simulink model "q_aero_2dof_pid_control_new"  (R2025a)
settings: Solver=ode1  StartTime=0.0  StopTime=Tend  FixedStep=0.002  RelTol=1e-3  EnableMultiTasking=on
PreLoadFcn:
  | quanser_aero_pd_design;
values from neighbouring files (symbols this model uses):
  kp_p = P.Jp*wp^2 - P.Ksp    [decoupled_pd_AERO.m]    (also in decoupled_pd_volt_torque.m = P.Jp*wn^2 - P.Ksp; figures_pd_presentation_AERO.m = P.Jp*wn^2 - P.Ksp; plot_decoupled_pd_tests_AERO.m = P.Jp*wn^2 - P.Ksp; setup_decoupled_pd_simulink.m = P.Jp*wn^2 - P.Ksp)
  kp_y = P.Jy*wy^2    [decoupled_pd_AERO.m]    (also in decoupled_pd_volt_torque.m = P.Jy*wn^2; figures_pd_presentation_AERO.m = P.Jy*wn^2; plot_decoupled_pd_tests_AERO.m = P.Jy*wn^2; setup_decoupled_pd_simulink.m = P.Jy*wn^2)
  Ksp = P.Ksp    [decoupled_pd_volt_torque.m]    (also in setup_decoupled_pd_simulink.m)
  W = inv(Wdec)    [decoupled_pd_AERO.m]    (also in decoupled_pd_volt_torque.m = inv([P.Kpp P.Kpy; P.Kyp P.Kyy]); setup_decoupled_pd_simulink.m = inv(Bt))
libraries: simulink_extras x4, quarc_library x3, quanser_aero x1
settings Model: SimulationMode=external  ExtModeTrigDuration=15000  Creator=MLevis  LastModifiedBy=e82540u
settings SolverCC: AlgebraicLoopSolver=TrustRegion  PositivePriorityOrder=on
settings DataIOCC: LimitDataPoints=on  SaveFormat=Array  ReturnWorkspaceOutputs=off
settings DebuggingCC: SolverPrmCheckMsg=warning  UnconnectedInputMsg=warning  UnconnectedOutputMsg=warning  UnconnectedLineMsg=warning  SFUnexpectedBacktrackingDiag=warning  SFNoUnconditionalDefaultTransitionDiag=warning  SFExecutionAtInitializationDiag=none  ArithmeticOperatorsInVariantConditions=warning
settings ModelReferenceCC: PropagateSignalLabelsOutOfModel=off
settings SFSimCC: SimUseLocalCustomCode=off  CustomCodeUndefinedFunction=UseInterfaceOnly
settings RTWCC: SystemTargetFile=quarc_win64.tlc  TemplateMakefile=quarc_default_tmf  RTWUseLocalCustomCode=off  Toolchain=QUARC win64 | nmake (64-bit Windows)  BuildConfiguration=Faster Runs  GPUComputeCapability=3.5  Description=QUARC Win64 Target Using Toolchain
settings CodeAppCC: StateflowObjectComments=on
settings STFCustomTargetCC: SystemTargetFile=quarc_win64.tlc  MultiwordLength=2048.0  DynamicStringBufferSize=256.0  ConcurrentExecutionCompliant=on  UseToolchainInfoCompliant=on
settings GRTTargetCC: ExtMode=on  ExtModeMexFile=quarc_comm  TargetLangStandard=C89/C90 (ANSI)  ParMdlRefBuildCompliant=off  CompOptLevelCompliant=off  CombineOutputUpdateFcns=off  MatFileLogging=off  CPPClassGenCompliant=off  GRTInterface=on
settings ConfigComp: CovMetricSettings=dw  CovSaveCumulativeToWorkspaceVar=on  CovSaveSingleToWorkspaceVar=on  CovExternalEMLEnable=off  CovSFcnEnable=off

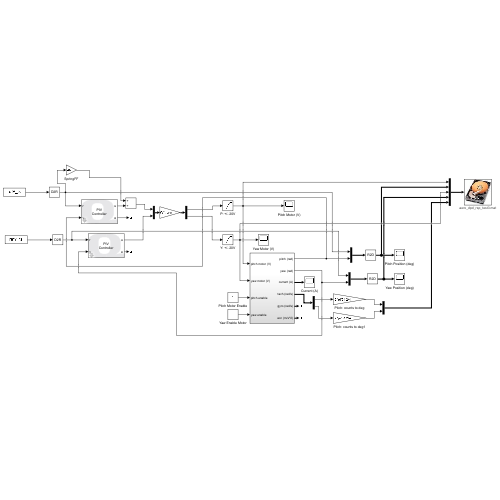
[thumbnail: Simulink's stored preview of the top-level diagram]
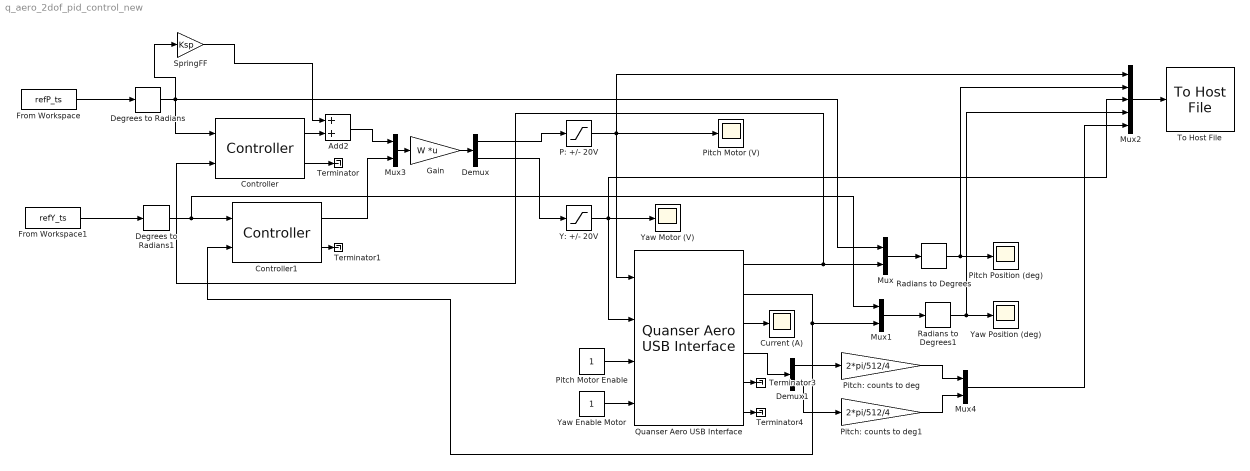
== system q_aero_2dof_pid_control_new ==
  Add2 : Sum
  Controller : quarc_library/Continuous/Controller  ctrl_type=Proportional-Integral-Velocity (PIV)  param_src=Specify via dialog  Kp=kp_p  Ki=0  Kd=0  Kv=kd_p  Ka=0  Wn=Wn_vel
      settings: SourceProductName=QUARC Targets
  Controller1 : quarc_library/Continuous/Controller  ctrl_type=Proportional-Integral-Velocity (PIV)  param_src=Specify via dialog  Kp=kp_y  Ki=0  Kd=0  Kv=kd_y  Ka=0  Wn=Wn_vel
      settings: SourceProductName=QUARC Targets
  Current (A) : Scope
      settings: TimeSpan=5  DataLoggingSaveFormat=Array
  Degrees to Radians : simulink_extras/Transformations/Degrees to Radians
  Degrees to Radians1 : simulink_extras/Transformations/Degrees to Radians
  Demux : Demux  Outputs=2
  Demux1 : Demux  Outputs=2
  From Workspace : FromWorkspace  VariableName=refP_ts  SampleTime=0.002  OutputAfterFinalValue=Holding final value
  From Workspace1 : FromWorkspace  VariableName=refY_ts  SampleTime=0.002  OutputAfterFinalValue=Holding final value
  Gain : Gain  Gain=W  Multiplication=Matrix(K*u) (u vector)
  Mux{,1,3..4} (4 alike) : Mux  Inputs=2
  Mux2 : Mux  Inputs=5
  P: +/- 20V : Saturate  UpperLimit=20  LowerLimit=-20
  Pitch Motor (V) : Scope
      settings: TimeSpan=30  ActiveDisplayYMinimum=-30  ActiveDisplayYMaximum=30  DataLoggingMaxPoints=15000  DataLoggingVariableName=ScopeData2  DataLoggingSaveFormat=Array
  Pitch Motor Enable : Constant
  Pitch Position (deg) : Scope
      settings: TimeSpan=30  ActiveDisplayYMinimum=-45  ActiveDisplayYMaximum=45  DataLoggingMaxPoints=15000  DataLoggingVariableName=ScopeData3  DataLoggingSaveFormat=Array
  Pitch: counts to deg : Gain  Gain=2*pi/512/4
  Pitch: counts to deg1 : Gain  Gain=2*pi/512/4
  Quanser Aero USB Interface : quanser_aero/Quanser Aero USB Interface  SystemSampleTime=-1  VariantActivationTime=update diagram  EmptyChoice=off  PassThrough=off  PassThroughVariantControl=(default)  EmptyChoiceVariantControl=(default)  AllowFlexibleInterface=on  Latency=0  AutoFrameSizeCalculation=off
  Radians to Degrees : simulink_extras/Transformations/Radians to Degrees
  Radians to Degrees1 : simulink_extras/Transformations/Radians to Degrees
  SpringFF : Gain  Gain=Ksp
  Terminator{,1,3..4} (4 alike) : Terminator
  To Host File : quarc_library/Sinks/To Host/To Host File  source=Specify via dialog (do not evaluate)  file_name=aero_dpd_rsp_test3.mat  variable_name=pid_rsp  decimation=1  sample_time=-1  file_format=MAT-file v.4  options=No header or footer  append=off  final_file_name=aero_dpd_rsp_test3.mat  encoding=Default  bitrate=0
  Y: +/- 20V : Saturate  UpperLimit=20  LowerLimit=-20
  Yaw Enable Motor : Constant
  Yaw Motor (V) : Scope
      settings: TimeSpan=30  ActiveDisplayYMinimum=-30  ActiveDisplayYMaximum=30  DataLoggingMaxPoints=15000  DataLoggingVariableName=ScopeData5  DataLoggingSaveFormat=Array
  Yaw Position (deg) : Scope
      settings: TimeSpan=30  ActiveDisplayYMinimum=-100  ActiveDisplayYMaximum=100  DataLoggingMaxPoints=15000  DataLoggingVariableName=ScopeData4  DataLoggingSaveFormat=Array
  wires:
  Quanser Aero USB Interface/3 -> Current (A)/1
  Quanser Aero USB Interface/1 -> Controller/2, Mux/2
  Degrees to Radians1/1 -> Controller1/1, Mux1/1
  Quanser Aero USB Interface/2 -> Controller1/2, Mux1/2
  Controller/2 -> Terminator/1
  Controller1/2 -> Terminator1/1
  From Workspace/1 -> Degrees to Radians/1
  From Workspace1/1 -> Degrees to Radians1/1
  Mux/1 -> Radians to Degrees/1
  Radians to Degrees/1 -> Mux2/2, Pitch Position (deg)/1
  Mux1/1 -> Radians to Degrees1/1
  Radians to Degrees1/1 -> Yaw Position (deg)/1, Mux2/4
  Pitch Motor Enable/1 -> Quanser Aero USB Interface/3
  Yaw Enable Motor/1 -> Quanser Aero USB Interface/4
  P: +/- 20V/1 -> Mux2/1, Quanser Aero USB Interface/1, Pitch Motor (V)/1
  Y: +/- 20V/1 -> Quanser Aero USB Interface/2, Mux2/3, Yaw Motor (V)/1
  Quanser Aero USB Interface/4 -> Demux1/1
  Quanser Aero USB Interface/5 -> Terminator3/1
  Quanser Aero USB Interface/6 -> Terminator4/1
  Mux2/1 -> To Host File/1
  SpringFF/1 -> Add2/1
  Degrees to Radians/1 -> Mux/1, Controller/1, SpringFF/1
  Controller/1 -> Add2/2
  Controller1/1 -> Mux3/2
  Add2/1 -> Mux3/1
  Mux3/1 -> Gain/1
  Gain/1 -> Demux/1
  Demux/1 -> P: +/- 20V/1
  Demux/2 -> Y: +/- 20V/1
  Demux1/1 -> Pitch: counts to deg/1
  Demux1/2 -> Pitch: counts to deg1/1
  Pitch: counts to deg/1 -> Mux4/1
  Pitch: counts to deg1/1 -> Mux4/2
  Mux4/1 -> Mux2/5
